simulink model "NonLinearVsStateSpace"  (R2025b)
settings: Solver=ode15s  StartTime=0.0  StopTime=10  RelTol=1e-3
PreLoadFcn:
  | Constants_and_state_space
undefined symbols (not defined in the file): A, B, C, CA_re, CAin_re, CB_re, D, QH_re, Qin_V_re, T_re, Tc_re, Tin_re
settings Model: Creator=Lenovo  LastModifiedBy=Lenovo

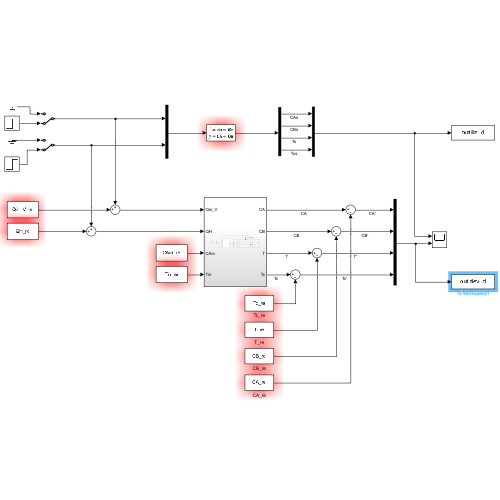
[thumbnail: Simulink's stored preview of the top-level diagram]
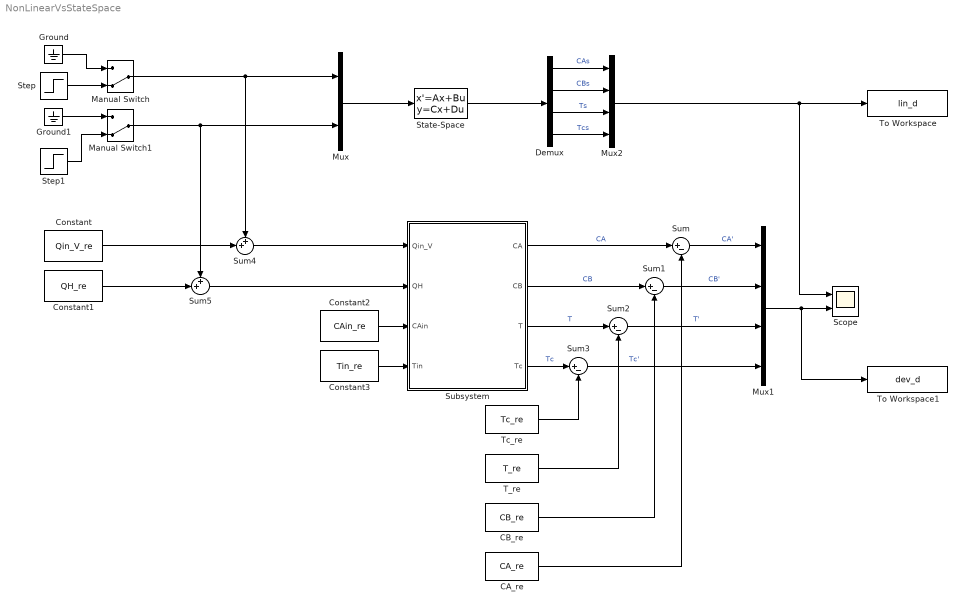
== system NonLinearVsStateSpace ==
  CA_re : Constant  Value=CA_re
  CB_re : Constant  Value=CB_re
  Constant : Constant  Value=Qin_V_re
  Constant1 : Constant  Value=QH_re
  Constant2 : Constant  Value=CAin_re
  Constant3 : Constant  Value=Tin_re
  Demux : Demux
  Ground : Ground
  Ground1 : Ground
  Manual Switch : ManualSwitch  CurrentSetting=0
  Manual Switch1 : ManualSwitch  CurrentSetting=0
  Mux : Mux  Inputs=2
  Mux1 : Mux
  Mux2 : Mux
  Scope : Scope  NumInputPorts=2
      settings: ActiveDisplayYMinimum=-9.2909293536014612  ActiveDisplayYMaximum=12.946724032775293
  State-Space : StateSpace  A=A  B=B  C=C  D=D  InitialCondition=0
  Step : Step  Time=5  SampleTime=0
  Step1 : Step  Time=5  SampleTime=0
  Subsystem : Subsystem
  Sum{,1..3} (4 alike) : Sum  Inputs=|+-
  Sum4 : Sum  Inputs=++|
  Sum5 : Sum  Inputs=++|
  T_re : Constant  Value=T_re
  Tc_re : Constant  Value=Tc_re
  To Workspace : ToWorkspace  VariableName=lin_d  SaveFormat=Structure With Time  SampleTime=-1
  To Workspace1 : ToWorkspace  VariableName=dev_d  SaveFormat=Structure With Time  SampleTime=-1
  wires:
  Mux/1 -> State-Space/1
  Subsystem/2(CB) -> Sum1/1  "CB"
  Constant3/1 -> Subsystem/4(Tin)
  Constant2/1 -> Subsystem/3(CAin)
  Subsystem/4(Tc) -> Sum3/1  "Tc"
  Subsystem/3(T) -> Sum2/1  "T"
  Subsystem/1(CA) -> Sum/1  "CA"
  Tc_re/1 -> Sum3/2
  T_re/1 -> Sum2/2
  CB_re/1 -> Sum1/2
  CA_re/1 -> Sum/2
  Sum/1 -> Mux1/1  "CA'"
  Sum1/1 -> Mux1/2  "CB'"
  Sum2/1 -> Mux1/3  "T'"
  Sum3/1 -> Mux1/4  "Tc'"
  Mux1/1 -> To Workspace1/1, Scope/2
  State-Space/1 -> Demux/1
  Demux/1 -> Mux2/1  "CAs"
  Demux/2 -> Mux2/2  "CBs"
  Demux/3 -> Mux2/3  "Ts"
  Demux/4 -> Mux2/4  "Tcs"
  Mux2/1 -> To Workspace/1, Scope/1
  Sum4/1 -> Subsystem/1(Qin_V)
  Constant/1 -> Sum4/2
  Sum5/1 -> Subsystem/2(QH)
  Constant1/1 -> Sum5/2
  Step/1 -> Manual Switch/2
  Manual Switch/1 -> Mux/1, Sum4/1
  Ground/1 -> Manual Switch/1
  Manual Switch1/1 -> Sum5/1, Mux/2
  Step1/1 -> Manual Switch1/2
  Ground1/1 -> Manual Switch1/1

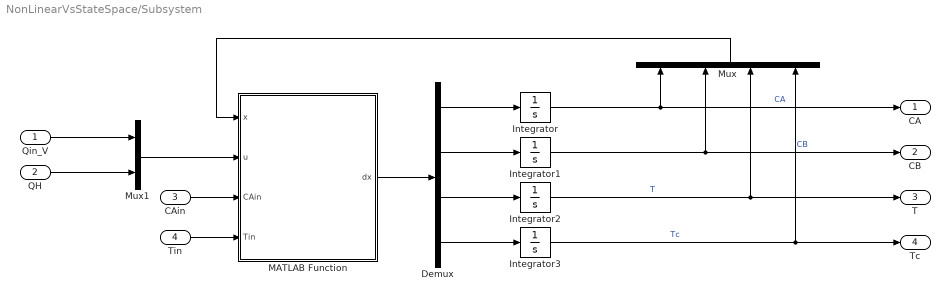
== system NonLinearVsStateSpace/Subsystem ==
  Qin_V : Inport
  QH : Inport  Port=2
  CAin : Inport  Port=3
  Tin : Inport  Port=4
  Demux : Demux
  Integrator : Integrator  InitialCondition=CA_re
  Integrator1 : Integrator  InitialCondition=CB_re
  Integrator2 : Integrator  InitialCondition=T_re
  Integrator3 : Integrator  InitialCondition=Tc_re
  MATLAB Function : MATLAB Function  TreatAsAtomicUnit=on
  Mux : Mux
  Mux1 : Mux  Inputs=2
  CA : Outport
  CB : Outport  Port=2
  T : Outport  Port=3
  Tc : Outport  Port=4
  wires:
  Demux/3 -> Integrator2/1
  Integrator1/1 -> CB/1, Mux/2  "CB"
  Integrator/1 -> CA/1, Mux/1  "CA"
  Mux/1 -> MATLAB Function/1(x)
  Integrator2/1 -> T/1, Mux/3  "T"
  Integrator3/1 -> Tc/1, Mux/4  "Tc"
  MATLAB Function/1(dx) -> Demux/1
  Demux/2 -> Integrator1/1
  Demux/4 -> Integrator3/1
  Demux/1 -> Integrator/1
  Mux1/1 -> MATLAB Function/2(u)
  Tin/1 -> MATLAB Function/4(Tin)
  QH/1 -> Mux1/2
  CAin/1 -> MATLAB Function/3(CAin)
  Qin_V/1 -> Mux1/1

== matlab function NonLinearVsStateSpace/Subsystem/MATLAB Function ==
  data: x input; u input; dx output; CAin input; Tin input
function dx = cstr_model(x, u, CAin, Tin)
dx = [0; 0; 0; 0]; 

% State variables

CA = x(1);
CB = x(2);
T  = x(3);
Tc = x(4);

% Manipulated variables
Qin_V = u(1);
QH    = u(2);

% Constants

V = 0.01;
Cp = 3.01;
den = 934.2; 
entAB = 4.2;
entBC = -11.0;
entAD = -41.85;
Ar = 0.215;
Kw = 4032;
mK = 5.0;
CpJ = 2.0;
k1_0 = 1.287e12;
k2_0 = 9.043e6;
E1 = -9758.3;
E2 = -8560.0;

% Arrhenius equations 

k1 = k1_0 * exp(E1 / (T + 273.15));
k2 = k2_0 * exp(E2 / (T + 273.15));

% Mass and energy balances

dx(1) = (Qin_V)*(CAin - CA) - k1*CA - k2*CA^2; % dCA/dt

dx(2) = -(Qin_V)*CB + k1*(CA - CB); %dCB/dt

dx(3) = (Qin_V)*(Tin - T) - (1/(den*Cp))*(k1*CA*entAB + k1*CB*entBC + k2*CA^2*entAD) + (Tc - T)*((Ar*Kw)/(den*Cp*V)); %dT/dt

dx(4) = (QH/(mK*CpJ)) + ((Ar*Kw)/(mK*CpJ))*(T - Tc); %dTc/dt

end
